simulink model "structure_track_shear"  (R2026b)
settings: Solver=VariableStepAuto
undefined symbols (not defined in the file or in its folder): P, Ts
settings Model: Creator=aomar  LastModifiedBy=aomar

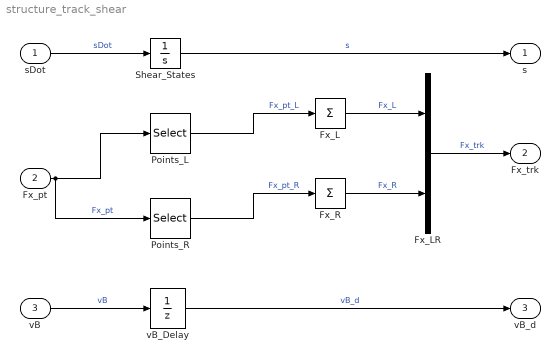
== system structure_track_shear ==
  sDot : Inport
  Fx_pt : Inport  Port=2
  vB : Inport  Port=3
  Fx_L : Sum  Inputs=+
  Fx_LR : Mux  Inputs=2
  Fx_R : Sum  Inputs=+
  Points_L : Selector  InputPortWidth=2*P.structure.track.Nc  IndexOptions=Index vector (dialog)  Indices=1:P.structure.track.Nc  OutputSizes=1
  Points_R : Selector  InputPortWidth=2*P.structure.track.Nc  IndexOptions=Index vector (dialog)  Indices=P.structure.track.Nc+1:2*P.structure.track.Nc  OutputSizes=1
  Shear_States : Integrator  InitialCondition=zeros(4*P.structure.track.Nc,1)  LimitOutput=on  UpperSaturationLimit=1  LowerSaturationLimit=-1  ZeroCross=off
  vB_Delay : UnitDelay  InitialCondition=P.structure.init.v0*[1;1]  SampleTime=Ts.base
  s : Outport
  Fx_trk : Outport  Port=2
  vB_d : Outport  Port=3
  wires:
  sDot/1 -> Shear_States/1  "sDot"
  Fx_pt/1 -> Points_L/1, Points_R/1  "Fx_pt"
  vB/1 -> vB_Delay/1  "vB"
  Shear_States/1 -> s/1  "s"
  vB_Delay/1 -> vB_d/1  "vB_d"
  Points_L/1 -> Fx_L/1  "Fx_pt_L"
  Points_R/1 -> Fx_R/1  "Fx_pt_R"
  Fx_L/1 -> Fx_LR/1  "Fx_L"
  Fx_R/1 -> Fx_LR/2  "Fx_R"
  Fx_LR/1 -> Fx_trk/1  "Fx_trk"
